simulink model "pid_standard"  (R2026b)
settings: Solver=ode4  StopTime=30  FixedStep=0.05
settings Model: Creator=ZAID  LastModifiedBy=ZAID

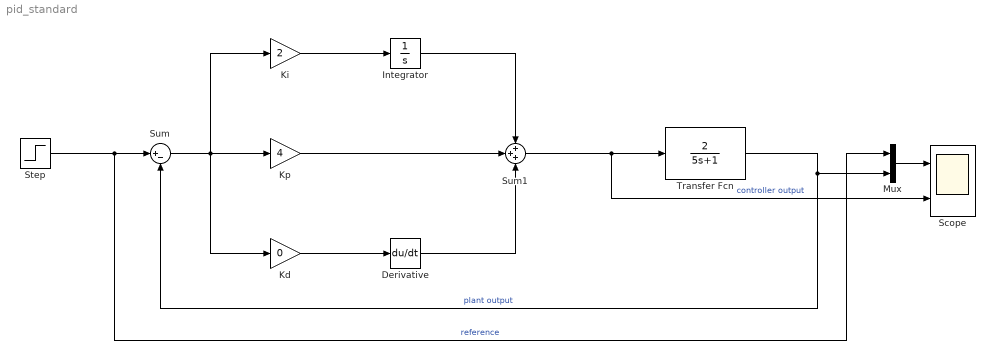
== system pid_standard ==
  Derivative : Derivative
  Integrator : Integrator
  Kd : Gain  Gain=0
  Ki : Gain  Gain=2
  Kp : Gain  Gain=4
  Mux : Mux  Inputs=2
  Scope : Scope  NumInputPorts=2
      settings: ActiveDisplayYMinimum=-2.0208029834285965  ActiveDisplayYMaximum=18.187226850857371
  Step : Step  FinalValue=15  SampleTime=0
  Sum : Sum  Inputs=|+-
  Sum1 : Sum  Inputs=+++
  Transfer Fcn : TransferFcn  Numerator=2  Denominator=[5 1]
  wires:
  Step/1 -> Sum/1, Mux/1  "reference"
  Sum/1 -> Ki/1, Kd/1, Kp/1
  Ki/1 -> Integrator/1
  Kd/1 -> Derivative/1
  Kp/1 -> Sum1/2
  Integrator/1 -> Sum1/1
  Derivative/1 -> Sum1/3
  Sum1/1 -> Transfer Fcn/1, Scope/2  "controller output"
  Transfer Fcn/1 -> Mux/2, Sum/2  "plant output"
  Mux/1 -> Scope/1
